simulink model "Termico_FP"  (R2022b)
settings: Solver=ode45  StartTime=0.0  StopTime=N-1  RelTol=1e-8  EnableMultiTasking=on
undefined symbols (not defined in the file): Ct, Ka, Kp, Kt, Kw, Ta, Td, Tp1, Tp2, Ts, Tz
settings Model: Creator=Adolfo  LastModifiedBy=adolfo
settings SolverCC: ZeroCrossControl=DisableAll  AlgebraicLoopSolver=TrustRegion
settings DataIOCC: LimitDataPoints=on  MaxDataPoints=25000  SaveFormat=Array  SignalLoggingSaveFormat=ModelDataLogs  ReturnWorkspaceOutputs=off
settings OptimizationCC: BlockReduction=off  BooleanDataType=off  ExpressionDepthLimit=2147483647  InitFltsAndDblsToZero=on  LifeSpan=inf
settings DebuggingCC: SaveWithParameterizedLinksMsg=none  UnderspecifiedInitializationDetection=Classic  MergeDetectMultiDrivingBlocksExec=none  SignalResolutionControl=TryResolveAllWithWarning  MultiTaskDSMMsg=warning  MultiTaskCondExecSysMsg=none  FcnCallInpInsideContextMsg=warning  UnconnectedInputMsg=warning  UnconnectedOutputMsg=warning  UnconnectedLineMsg=warning  StateNameClashWarn=warning  SFUnexpectedBacktrackingDiag=warning  SFNoUnconditionalDefaultTransitionDiag=warning  SFExecutionAtInitializationDiag=none  SFMachineParentedDataDiag=warning  ArithmeticOperatorsInVariantConditions=warning
settings HardwareCC: ProdBitPerPointer=32  ProdBitPerSizeT=32  ProdBitPerPtrDiffT=32  ProdLargestAtomicFloat=None  ProdIntDivRoundTo=Undefined  ProdEndianess=Unspecified  ProdWordSize=32  ProdHWDeviceType=32-bit Generic  TargetUnknown=on
settings ModelReferenceCC: EnableRefExpFcnMdlSchedulingChecks=on  PropagateSignalLabelsOutOfModel=off
settings SFSimCC: SimUseLocalCustomCode=off  CustomCodeUndefinedFunction=UseInterfaceOnly
settings RTWCC: RTWUseLocalCustomCode=off
settings CodeAppCC: StateflowObjectComments=on
settings GRTTargetCC: TargetFcnLib=ansi_tfl_tmw.mat  TargetLangStandard=C89/C90 (ANSI)  CombineOutputUpdateFcns=off  GRTInterface=on
settings ConfigComp: CovMetricSettings=dw  CovSaveCumulativeToWorkspaceVar=on  CovSaveSingleToWorkspaceVar=on  CovExternalEMLEnable=off

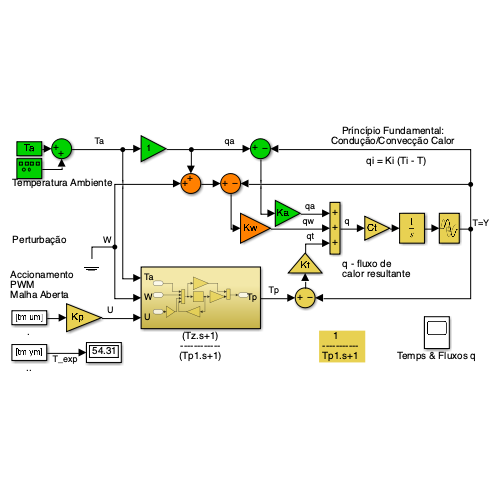
[thumbnail: Simulink's stored preview of the top-level diagram]
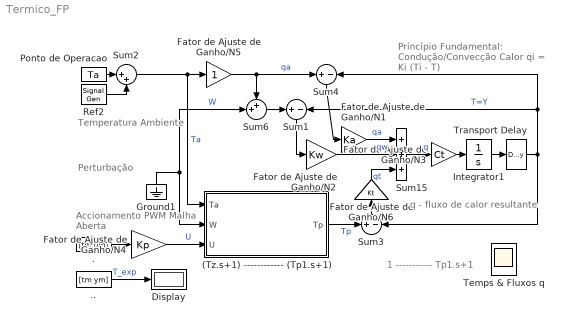
== system Termico_FP ==
  note: Accionamento
      | PWM
      | Malha Aberta
  note: Perturbação
  note: Príncípio Fundamental:
      | Condução/Convecção Calor
      |
      |              qi = Ki (Ti - T)
  note: 1
      |  -----------
      |  Tp1.s+1
  note: q - fluxo de
      | calor resultante
  note: Temperatura Ambiente
  (Tz.s+1) ------------ (Tp1.s+1) : Subsystem
  . : FromWorkspace  VariableName=[tm um]  SampleTime=Ts
  .. : FromWorkspace  VariableName=[tm ym]  SampleTime=Ts
  Display : Display
  Fator de Ajuste de Ganho/N1 : Gain  Gain=Ka  SaturateOnIntegerOverflow=on  OutDataTypeStr=Inherit: Same as input  ParamDataTypeStr=Inherit: Same as input
  Fator de Ajuste de Ganho/N2 : Gain  Gain=Kw  SaturateOnIntegerOverflow=on  OutDataTypeStr=Inherit: Same as input  ParamDataTypeStr=Inherit: Same as input
  Fator de Ajuste de Ganho/N3 : Gain  Gain=Ct  SaturateOnIntegerOverflow=on  OutDataTypeStr=Inherit: Same as input  ParamDataTypeStr=Inherit: Same as input
  Fator de Ajuste de Ganho/N4 : Gain  Gain=Kp  SaturateOnIntegerOverflow=on  OutDataTypeStr=Inherit: Same as input  ParamDataTypeStr=Inherit: Same as input
  Fator de Ajuste de Ganho/N5 : Gain  SaturateOnIntegerOverflow=on  OutDataTypeStr=Inherit: Same as input  ParamDataTypeStr=Inherit: Same as input
  Fator de Ajuste de Ganho/N6 : Gain  Gain=Kt  SaturateOnIntegerOverflow=on  OutDataTypeStr=Inherit: Same as input  ParamDataTypeStr=Inherit: Same as input
  Ground1 : Ground
  Integrator1 : Integrator  InitialCondition=Ta
  Ponto de Operacao : Constant  Value=Ta
  Ref2 : SignalGenerator  Amplitude=2  Frequency=1/3600/24
  Sum1 : Sum  Inputs=+|-  InputSameDT=on  SaturateOnIntegerOverflow=on  OutDataTypeStr=Inherit: Same as first input
  Sum15 : Sum  Inputs=+++  InputSameDT=on  SaturateOnIntegerOverflow=on  OutDataTypeStr=Inherit: Same as first input
  Sum2 : Sum  Inputs=|++
  Sum3 : Sum  Inputs=+|-  InputSameDT=on  SaturateOnIntegerOverflow=on  OutDataTypeStr=Inherit: Same as first input
  Sum4 : Sum  Inputs=+|-  InputSameDT=on  SaturateOnIntegerOverflow=on  OutDataTypeStr=Inherit: Same as first input
  Sum6 : Sum  Inputs=++|
  Temps & Fluxos q : Scope
      settings: Floating=on
  Transport Delay : TransportDelay  DelayTime=Td  InitialOutput=Ta  BufferSize=2048  PadeOrder=2
  wires:
  Sum15/1 -> Fator de Ajuste de Ganho/N3/1  "q"
  Fator de Ajuste de Ganho/N3/1 -> Integrator1/1
  Sum3/1 -> Fator de Ajuste de Ganho/N6/1
  Fator de Ajuste de Ganho/N4/1 -> (Tz.s+1) ------------ (Tp1.s+1)/3(U)  "U"
  Transport Delay/1 -> Sum3/2, Sum1/2, Sum4/2  "T=Y"
  (Tz.s+1) ------------ (Tp1.s+1)/1(Tp) -> Sum3/1  "Tp"
  Fator de Ajuste de Ganho/N6/1 -> Sum15/3  "qt"
  Ponto de Operacao/1 -> Sum2/1
  Sum1/1 -> Fator de Ajuste de Ganho/N2/1
  Integrator1/1 -> Transport Delay/1
  Ground1/1 -> (Tz.s+1) ------------ (Tp1.s+1)/2(W), Sum6/2  "W"
  Fator de Ajuste de Ganho/N2/1 -> Sum15/2  "qw"
  ./1 -> Fator de Ajuste de Ganho/N4/1
  Sum4/1 -> Fator de Ajuste de Ganho/N1/1
  Fator de Ajuste de Ganho/N1/1 -> Sum15/1  "qa"
  Sum6/1 -> Sum1/1
  ../1 -> Display/1  "T_exp"
  Ref2/1 -> Sum2/2
  Sum2/1 -> Fator de Ajuste de Ganho/N5/1, (Tz.s+1) ------------ (Tp1.s+1)/1(Ta)  "Ta"
  Fator de Ajuste de Ganho/N5/1 -> Sum6/1, Sum4/1  "qa"

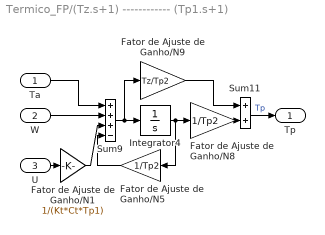
== system Termico_FP/(Tz.s+1) ------------ (Tp1.s+1) ==
  Ta : Inport
  W : Inport  Port=2
  U : Inport  Port=3
  Fator de Ajuste de Ganho/N1 : Gain  Gain=1/(Kt*Ct*Tp1)  SaturateOnIntegerOverflow=on  OutDataTypeStr=Inherit: Same as input  ParamDataTypeStr=Inherit: Same as input
  Fator de Ajuste de Ganho/N5 : Gain  Gain=1/Tp2  SaturateOnIntegerOverflow=on  OutDataTypeStr=Inherit: Same as input  ParamDataTypeStr=Inherit: Same as input
  Fator de Ajuste de Ganho/N8 : Gain  Gain=1/Tp2  SaturateOnIntegerOverflow=on  OutDataTypeStr=Inherit: Same as input  ParamDataTypeStr=Inherit: Same as input
  Fator de Ajuste de Ganho/N9 : Gain  Gain=Tz/Tp2  SaturateOnIntegerOverflow=on  OutDataTypeStr=Inherit: Same as input  ParamDataTypeStr=Inherit: Same as input
  Integrator4 : Integrator  InitialCondition=Ta*Tp2
  Sum11 : Sum  InputSameDT=on  SaturateOnIntegerOverflow=on  OutDataTypeStr=Inherit: Same as first input
  Sum9 : Sum  Inputs=+++-
  Tp : Outport
  wires:
  Ta/1 -> Sum9/1
  Fator de Ajuste de Ganho/N5/1 -> Sum9/4
  Sum11/1 -> Tp/1  "Tp"
  U/1 -> Fator de Ajuste de Ganho/N1/1
  Fator de Ajuste de Ganho/N9/1 -> Sum11/1
  Fator de Ajuste de Ganho/N8/1 -> Sum11/2
  W/1 -> Sum9/2
  Sum9/1 -> Fator de Ajuste de Ganho/N9/1, Integrator4/1
  Integrator4/1 -> Fator de Ajuste de Ganho/N8/1, Fator de Ajuste de Ganho/N5/1
  Fator de Ajuste de Ganho/N1/1 -> Sum9/3
